simulink library "pgmanif"  (R2016b)
settings: Solver=VariableStepAuto  StartTime=0.0  StopTime=10.0  RelTol=1e-3
settings Model: Creator=Maximilian  LastModifiedBy=mueh_mm
settings OptimizationCC: LifeSpan=inf
settings DebuggingCC: SFExecutionAtInitializationDiag=none

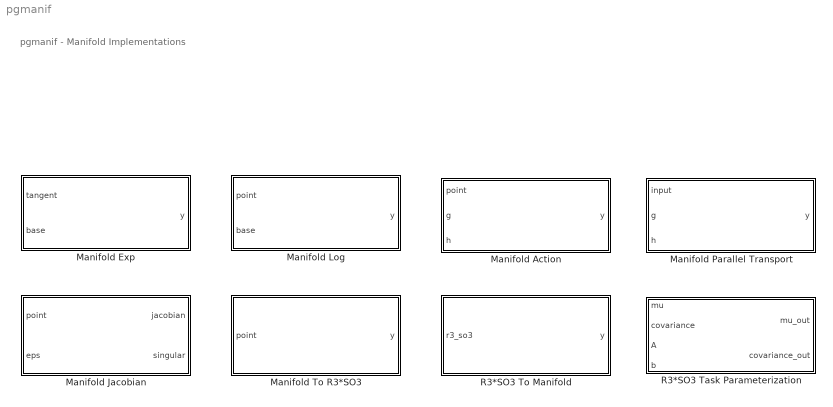
== system pgmanif ==
  note: pgmanif - Manifold Implementations
  Manifold Action : MATLAB Function  TreatAsAtomicUnit=on  mask(Manifold Action){manifold_description_raw=SO2, manifold_description=0, dim_manifold=0, dim_tangent=0}
      mask prompts: manifold_description_raw "Manifold Description"
      mask help: This block performs the manifold action, moving point defined relative to g to the same relative location of h.
      mask init:
      | % mask setup
      | mask_styles = get_param(gcb, 'MaskStyles');
      | mask_styles{1} = get_manifold_popup();
      | set_param(gcb, 'MaskStyles', mask_styles);
      | 
      | % set description
      | manifold_description = uint8(manifold_description_raw);
      | [dim_manifold, dim_tangent, ~] = pglfd.manif.util.get_manifold_dim_id(char(manifold_description));
  Manifold Exp : MATLAB Function  TreatAsAtomicUnit=on  mask(Manifold Exponential){manifold_description_raw=S2*R1*SO3, manifold_description=0, dim_manifold=0, dim_tangent=0}
      mask prompts: manifold_description_raw "Manifold Description"
      mask help: This block calculates the manifold exponential of tangent at base.
      mask init: same as pgmanif/Manifold Action
  Manifold Jacobian : MATLAB Function  TreatAsAtomicUnit=on  mask(Manifold Jacobian){manifold_description_raw=SO2, manifold_description=0, dim_manifold=0, dim_tangent=0, manifold_id=0}
      mask prompts: manifold_description_raw "Manifold Description"
      mask help: This block calculates the manifold jacobian at point. For a radius < eps, the corresponding entries are set to zero.
      mask init:
      | % mask setup
      | mask_styles = get_param(gcb, 'MaskStyles');
      | mask_styles{1} = get_manifold_popup();
      | set_param(gcb, 'MaskStyles', mask_styles);
      | 
      | % set description
      | manifold_description = uint8(manifold_description_raw);
      | [dim_manifold, dim_tangent, manifold_id] = pglfd.manif.util.get_manifold_dim_id(char(manifold_description));
  Manifold Log : MATLAB Function  TreatAsAtomicUnit=on  mask(Manifold Logarithm){manifold_description_raw=SO3, manifold_description=0, dim_manifold=0, dim_tangent=0}
      mask prompts: manifold_description_raw "Manifold Description"
      mask help: This block calculates the manifold logarithm of point at base.
      mask init: same as pgmanif/Manifold Action
  Manifold Parallel Transport : MATLAB Function  TreatAsAtomicUnit=on  mask(Manifold Parallel Transport){manifold_description_raw=SO2, manifold_description=0, dim_manifold=0, dim_tangent=0}
      mask prompts: manifold_description_raw "Manifold Description"
      mask help: This block parallel transports input (tangent vector or tangent matrix) from the manifold element g to the manifold element h.
      mask init: same as pgmanif/Manifold Action
  Manifold To R3*SO3 : MATLAB Function  TreatAsAtomicUnit=on  mask(Manifold To R3*SO3){manifold_description_raw=SO2, manifold_description=0, dim_manifold=0, dim_tangent=0}
      mask prompts: manifold_description_raw "Manifold Description"
      mask help: This block calculates the manifold element corresponding to the given R3*SO3 pose.
      mask init: same as pgmanif/Manifold Action
  R3*SO3 Task Parameterization : MATLAB Function  TreatAsAtomicUnit=on  mask(Manifold Task Parametrization){manifold_description=, dim_tangent=0, dim_manifold=0}
      mask help: This block performs task parametrization, Au + b on the R3*SO3 manifold. A is a transformation (rotation) and b a translation.
      mask init:
      | % set description
      | manifold_description = uint8('R3*SO3');
      | [dim_manifold, dim_tangent, ~] = pglfd.manif.util.get_manifold_dim_id(char(manifold_description));
  R3*SO3 To Manifold : MATLAB Function  TreatAsAtomicUnit=on  mask(R3*SO3 To Manifold){manifold_description_raw=SO2, manifold_description=0, dim_manifold=0, dim_tangent=0}
      mask prompts: manifold_description_raw "Manifold Description"
      mask help: This block calculates the R3*SO3 pose corresponding to the given manifold element.
      mask init: same as pgmanif/Manifold Action

== matlab function pgmanif/Manifold Action ==
  data: point input; g input; h input; y output; manifold_description parameter uint8; dim_manifold parameter; dim_tangent parameter
function y = fcn(point, g, h, manifold_description, dim_manifold, dim_tangent)

persistent manifold;
if isempty(manifold)
    manifold = pglfd.manif.util.get_productmanifold(char(manifold_description), dim_manifold, dim_tangent);
end

y = manifold.action(point, g, h);

== matlab function pgmanif/Manifold Log ==
  data: point input; base input; y output; manifold_description parameter uint8; dim_manifold parameter; dim_tangent parameter
function y = fcn(point, base, manifold_description, dim_manifold, dim_tangent)

persistent manifold;
if isempty(manifold)
    manifold = pglfd.manif.util.get_productmanifold(char(manifold_description), dim_manifold, dim_tangent);
end

y = manifold.log(point, base);

== matlab function pgmanif/Manifold Parallel Transport ==
  data: input input; g input; y output; manifold_description parameter uint8; dim_manifold parameter; dim_tangent parameter; h input
function y = fcn(input, g, manifold_description, dim_manifold, dim_tangent, h)

persistent manifold;
if isempty(manifold)
    manifold = pglfd.manif.util.get_productmanifold(char(manifold_description), dim_manifold, dim_tangent);
end

y = manifold.parallel_transport(input, g, h);

== matlab function pgmanif/Manifold Exp ==
  data: tangent input; base input; y output; manifold_description parameter uint8; dim_manifold parameter; dim_tangent parameter
function y = fcn(tangent, base, manifold_description, dim_manifold, dim_tangent)

persistent manifold;
if isempty(manifold)
    manifold = pglfd.manif.util.get_productmanifold(char(manifold_description), dim_manifold, dim_tangent);
end

y = manifold.exp(tangent, base);

== matlab function pgmanif/Manifold Jacobian ==
  data: point input; eps input; jacobian output; manifold_description parameter uint8; dim_manifold parameter; dim_tangent parameter; manifold_id parameter; singular output
function [jacobian, singular] = fcn(point, eps, manifold_description, dim_manifold, dim_tangent, manifold_id)

persistent manifold;
if isempty(manifold)
    manifold = pglfd.manif.util.get_productmanifold(char(manifold_description), dim_manifold, dim_tangent);
end

[jacobian, singular] = pglfd.manif.jacobian.manifold_jacobian_by_id(manifold_id, manifold, point, eps);

== matlab function pgmanif/Manifold To R3*SO3 ==
  data: point input; y output; manifold_description parameter uint8; dim_manifold parameter; dim_tangent parameter
function y = fcn(point, manifold_description, dim_manifold, dim_tangent)

persistent manifold;
if isempty(manifold)
    manifold = pglfd.manif.util.get_productmanifold(char(manifold_description), dim_manifold, dim_tangent);
end

y = pglfd.manif.conversions.manifold_to_r3_so3(manifold, point);

== matlab function pgmanif/R3*SO3 To Manifold ==
  data: r3_so3 input; y output; manifold_description parameter uint8; dim_manifold parameter; dim_tangent parameter
function y = fcn(r3_so3, manifold_description, dim_manifold, dim_tangent)

persistent manifold;
if isempty(manifold)
    manifold = pglfd.manif.util.get_productmanifold(char(manifold_description), dim_manifold, dim_tangent);
end

y = pglfd.manif.conversions.manifold_from_r3_so3(manifold, r3_so3);

== matlab function pgmanif/R3*SO3 Task Parameterization ==
  data: mu input; covariance input; A input; b input; mu_out output; manifold_description parameter uint8; dim_manifold parameter; dim_tangent parameter; covariance_out output size=[6,6]
function [mu_out, covariance_out] = fcn(mu, covariance, A, b, manifold_description, dim_manifold, dim_tangent)

persistent manifold;
if isempty(manifold)
    manifold = pglfd.manif.util.get_productmanifold(char(manifold_description), dim_manifold, dim_tangent);
end

mu_out = manifold.exp(A*manifold.log(mu,manifold.id_element),b);
covariance_out = A*covariance*A';
% TODO in the S2 case, this parallel transport is needed
%covariance_out = manifold.parallel_transport(covariance_out,b,mu_out);
